simulink model "orig_exp_i"  (R2023a)
settings: Solver=ode4  StartTime=0.0  StopTime=10  FixedStep=0.001  RelTol=1e-3
settings Model: Creator=Anonymous  LastModifiedBy=Anonymous

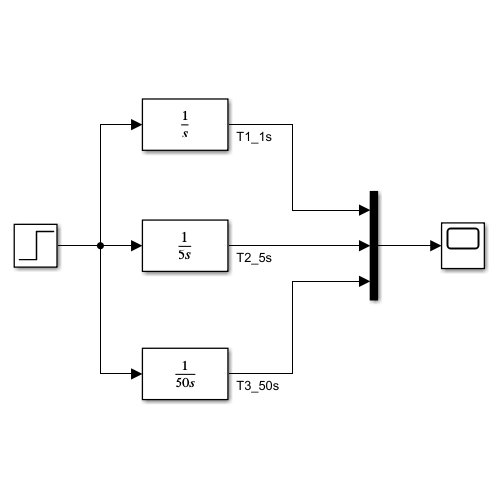
[thumbnail: Simulink's stored preview of the top-level diagram]
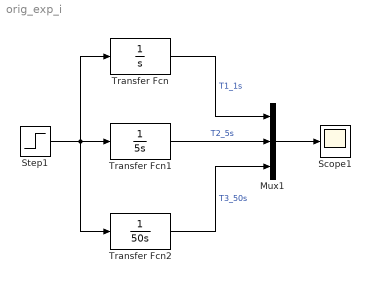
== system orig_exp_i ==
  Mux1 : Mux  Inputs=3
  Scope1 : Scope
  Step1 : Step  SampleTime=0
  Transfer Fcn : TransferFcn  Numerator=1  Denominator=[1 0]
  Transfer Fcn1 : TransferFcn  Numerator=1  Denominator=[5 0]
  Transfer Fcn2 : TransferFcn  Numerator=1  Denominator=[50 0]
  wires:
  Mux1/1 -> Scope1/1
  Transfer Fcn2/1 -> Mux1/3  "T3_50s"
  Transfer Fcn1/1 -> Mux1/2  "T2_5s"
  Transfer Fcn/1 -> Mux1/1  "T1_1s"
  Step1/1 -> Transfer Fcn2/1, Transfer Fcn1/1, Transfer Fcn/1
